simulink model "Algorithm"  (R2024a)
settings: Solver=FixedStepDiscrete  StartTime=0.0  StopTime=ALG_Stop_Time  FixedStep=ALG_Step_Size  RelTol=1e-3  EnableMultiTasking=on
undefined symbols (not defined in the file): BSD_WARN_DISTANCE_M, BSDState_T, RadarStatus_T, SignalStatus_T, TurnSignal_T, VSPD_SUPPRESSION_THRESHOLD
libraries: simulink x14
settings Model: DataDictionary=bsd.sldd  Creator=pc  LastModifiedBy=pc
settings OptimizationCC: DefaultParameterBehavior=Inlined  UseDivisionForNetSlopeComputation=on  EnhancedBackFolding=on  PassReuseOutputArgsAs=Individual arguments  ZeroExternalMemoryAtStartup=off  ZeroInternalMemoryAtStartup=off  OptimizeBlockOrder=speed  DifferentSizesBufferReuse=on  OptimizationCustomize=off  EfficientTunableParamExpr=on
settings DebuggingCC: ParameterTunabilityLossMsg=error
settings SFSimCC: MATLABDynamicMemAlloc=off
settings RTWCC: Description=AUTOSAR  SystemTargetFile=autosar.tlc  GenCodeOnly=on  TemplateMakefile=ert_default_tmf  DataTypeReplacement=CDataTypesFixedWidth
settings CodeAppCC: ForceParamTrailComments=on  IgnoreCustomStorageClasses=off  OperatorAnnotations=on  SimulinkDataObjDesc=on  SFDataObjDesc=on  InsertBlockDesc=on
settings STFCustomTargetCC: MultiwordLength=256  ParMdlRefBuildCompliant=on  CompOptLevelCompliant=on  IncludeMdlTerminateFcn=off  CombineOutputUpdateFcns=on  SuppressErrorStatus=on  ERTCustomFileBanners=on  SupportNonFinite=off  SupportComplex=off  SupportContinuousTime=off  SupportNonInlinedSFcns=off  RemoveResetFunc=on  MATLABClassNameForMDSCustomization=Simulink.SoftwareTarget.ERTCustomization  AutosarCompliant=on  GRTInterface=off  LookupTableObjectStructAxisOrder=2,1,3,4,...  LUTObjectStructOrderEvenSpacing=Size,Table,Breakpoints  SystemTargetFile=autosar.tlc
settings ERTTargetCC: TargetLangStandard=C99 (ISO)  ConcurrentExecutionCompliant=off  IncludeMdlTerminateFcn=off  SuppressErrorStatus=on  SupportNonFinite=off  SupportComplex=off  ModelStepFunctionPrototypeControlCompliant=off  CPPClassGenCompliant=off  AutosarCompliant=on  LookupTableObjectStructAxisOrder=2,1,3,4,...  LUTObjectStructOrderEvenSpacing=Size,Table,Breakpoints  InlinedParameterPlacement=NonHierarchical  ERTCustomFileTemplate=example_file_process.tlc  BooleanTrueId=TRUE  BooleanFalseId=FALSE

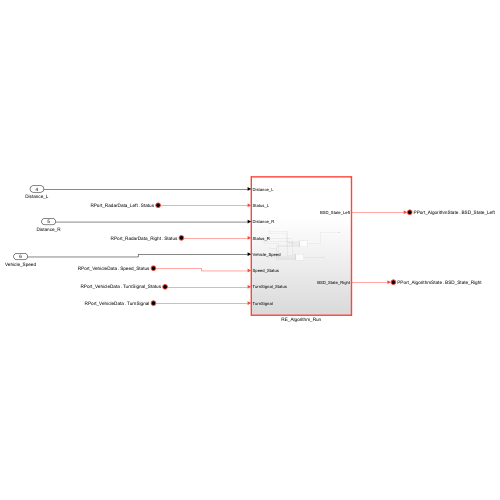
[thumbnail: Simulink's stored preview of the top-level diagram]
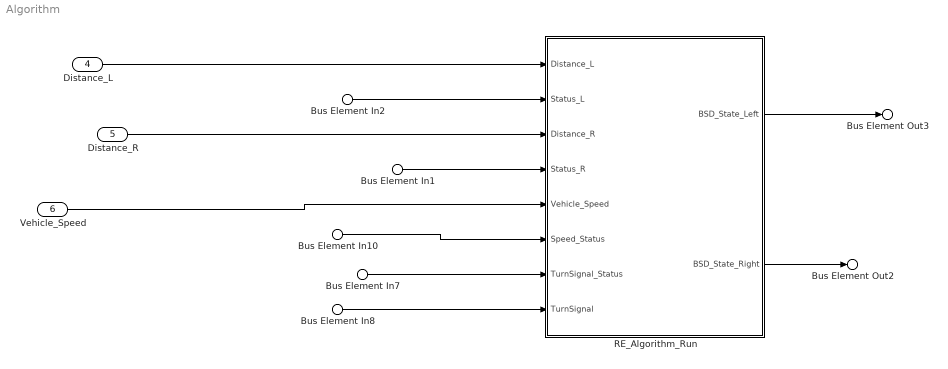
== system Algorithm ==
  Bus Element In7 : Inport  PortName=RPort_VehicleData  Element=TurnSignal_Status
  Bus Element In8 : Inport  PortName=RPort_VehicleData  Element=TurnSignal
  Bus Element In10 : Inport  PortName=RPort_VehicleData  Element=Speed_Status
  Bus Element In1 : Inport  Port=2  PortName=RPort_RadarData_Right  Element=Status
  Bus Element In2 : Inport  Port=3  PortName=RPort_RadarData_Left  Element=Status
  Distance_L : Inport  Port=4  OutDataTypeStr=Distance_m_T
  Distance_R : Inport  Port=5  OutDataTypeStr=Distance_m_T
  Vehicle_Speed : Inport  Port=6  OutDataTypeStr=Vehicle_Speed_T
  RE_Algorithm_Run : Subsystem  TreatAsAtomicUnit=on
  Bus Element Out2 : Outport  PortName=PPort_AlgorithmState  Element=BSD_State_Right
  Bus Element Out3 : Outport  PortName=PPort_AlgorithmState  Element=BSD_State_Left
  wires:
  Vehicle_Speed/1 -> RE_Algorithm_Run/5(Vehicle_Speed)
  Bus Element In10/1 -> RE_Algorithm_Run/6(Speed_Status)
  Bus Element In1/1 -> RE_Algorithm_Run/4(Status_R)
  Distance_L/1 -> RE_Algorithm_Run/1(Distance_L)
  Bus Element In2/1 -> RE_Algorithm_Run/2(Status_L)
  Distance_R/1 -> RE_Algorithm_Run/3(Distance_R)
  RE_Algorithm_Run/2(BSD_State_Right) -> Bus Element Out2/1
  RE_Algorithm_Run/1(BSD_State_Left) -> Bus Element Out3/1
  Bus Element In8/1 -> RE_Algorithm_Run/8(TurnSignal)
  Bus Element In7/1 -> RE_Algorithm_Run/7(TurnSignal_Status)

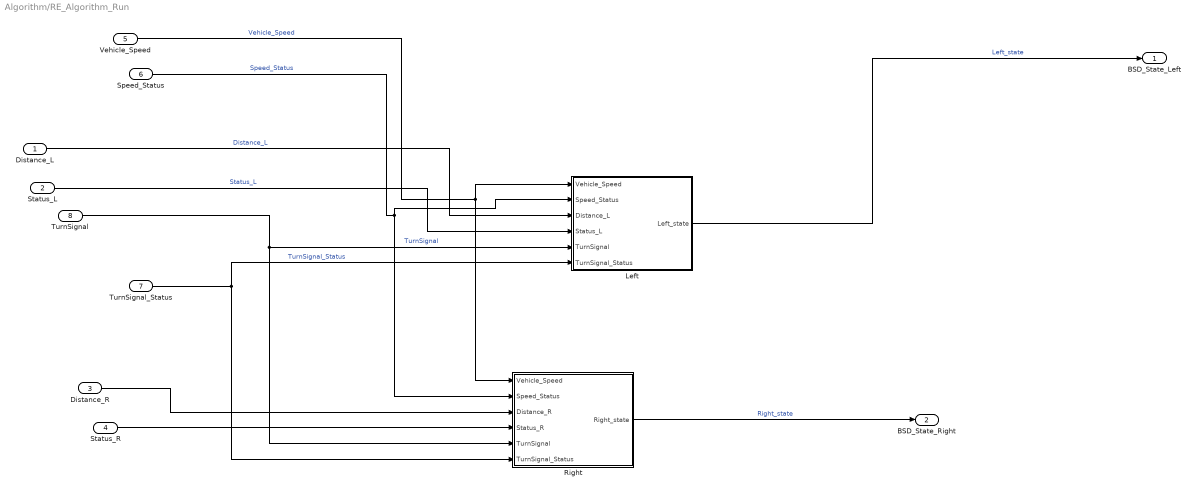
== system Algorithm/RE_Algorithm_Run ==
  Distance_L : Inport  OutDataTypeStr=Distance_m_T
  Status_L : Inport  Port=2  OutDataTypeStr=Enum: RadarStatus_T
  Distance_R : Inport  Port=3  OutDataTypeStr=Distance_m_T
  Status_R : Inport  Port=4  OutDataTypeStr=Enum: RadarStatus_T
  Vehicle_Speed : Inport  Port=5  OutDataTypeStr=Vehicle_Speed_T
  Speed_Status : Inport  Port=6  OutDataTypeStr=Enum: SignalStatus_T
  TurnSignal_Status : Inport  Port=7  OutDataTypeStr=Enum: SignalStatus_T
  TurnSignal : Inport  Port=8  OutDataTypeStr=Enum: TurnSignal_T
  Left : Subsystem
  Right : Subsystem
  BSD_State_Left : Outport  OutDataTypeStr=Enum: BSDState_T
  BSD_State_Right : Outport  Port=2  OutDataTypeStr=Enum: BSDState_T
  wires:
  Vehicle_Speed/1 -> Right/1(Vehicle_Speed), Left/1(Vehicle_Speed)  "Vehicle_Speed"
  Speed_Status/1 -> Right/2(Speed_Status), Left/2(Speed_Status)  "Speed_Status"
  Distance_L/1 -> Left/3(Distance_L)  "Distance_L"
  Status_L/1 -> Left/4(Status_L)  "Status_L"
  TurnSignal/1 -> Right/5(TurnSignal), Left/5(TurnSignal)  "TurnSignal"
  TurnSignal_Status/1 -> Left/6(TurnSignal_Status), Right/6(TurnSignal_Status)  "TurnSignal_Status"
  Left/1(Left_state) -> BSD_State_Left/1  "Left_state"
  Right/1(Right_state) -> BSD_State_Right/1  "Right_state"
  Distance_R/1 -> Right/3(Distance_R)
  Status_R/1 -> Right/4(Status_R)

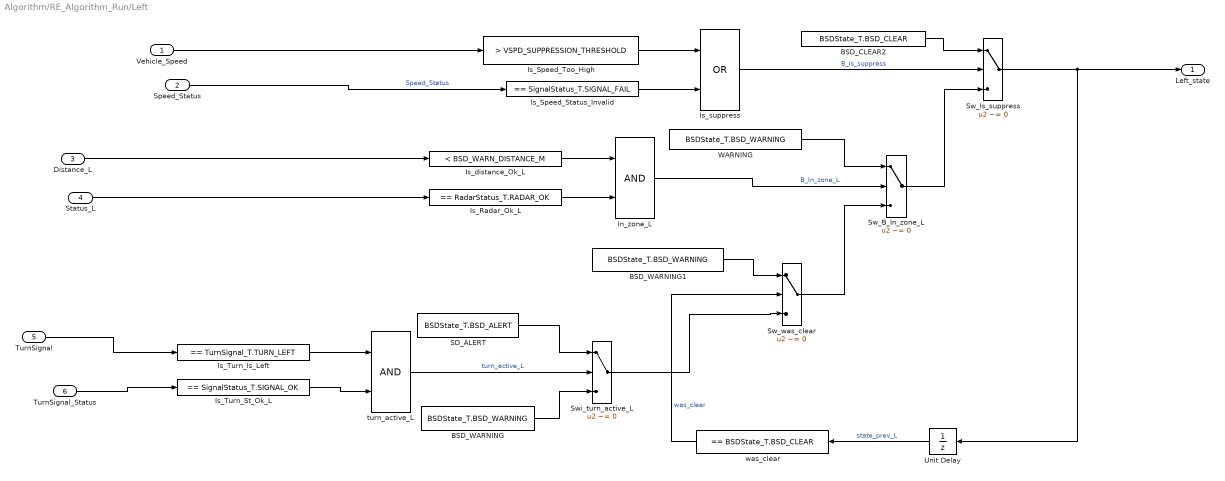
== system Algorithm/RE_Algorithm_Run/Left ==
  Vehicle_Speed : Inport  OutDataTypeStr=Vehicle_Speed_T
  Speed_Status : Inport  Port=2
  Distance_L : Inport  Port=3  OutDataTypeStr=Distance_m_T
  Status_L : Inport  Port=4
  TurnSignal : Inport  Port=5
  TurnSignal_Status : Inport  Port=6
  BSD_CLEAR2 : Constant  Value=BSDState_T.BSD_CLEAR  OutDataTypeStr=Enum: BSDState_T
  BSD_WARNING : Constant  Value=BSDState_T.BSD_WARNING  OutDataTypeStr=Enum: BSDState_T
  BSD_WARNING1 : Constant  Value=BSDState_T.BSD_WARNING  OutDataTypeStr=Enum: BSDState_T
  In_zone_L : Logic  AllPortsSameDT=off  OutDataTypeStr=boolean
  Is_Radar_Ok_L : simulink/Logic and Bit Operations/Compare To Constant  relop===  const=RadarStatus_T.RADAR_OK  OutDataTypeStr=boolean
  Is_Speed_Status_Invalid : simulink/Logic and Bit Operations/Compare To Constant  relop===  const=SignalStatus_T.SIGNAL_FAIL  OutDataTypeStr=boolean
  Is_Speed_Too_High : simulink/Logic and Bit Operations/Compare To Constant  relop=>  const=VSPD_SUPPRESSION_THRESHOLD  OutDataTypeStr=boolean
  Is_Turn_Is_Left : simulink/Logic and Bit Operations/Compare To Constant  relop===  const=TurnSignal_T.TURN_LEFT  OutDataTypeStr=boolean
  Is_Turn_St_Ok_L : simulink/Logic and Bit Operations/Compare To Constant  relop===  const=SignalStatus_T.SIGNAL_OK  OutDataTypeStr=boolean
  Is_distance_Ok_L : simulink/Logic and Bit Operations/Compare To Constant  relop=<  const=BSD_WARN_DISTANCE_M  OutDataTypeStr=boolean
  Is_suppress : Logic  Operator=OR  AllPortsSameDT=off  OutDataTypeStr=boolean
  SD_ALERT : Constant  Value=BSDState_T.BSD_ALERT  OutDataTypeStr=Enum: BSDState_T
  Sw_B_In_zone_L : Switch  Criteria=u2 ~= 0  SaturateOnIntegerOverflow=off  InputSameDT=off
  Sw_Is_suppress : Switch  Criteria=u2 ~= 0  SaturateOnIntegerOverflow=off  InputSameDT=off
  Sw_was_clear : Switch  Criteria=u2 ~= 0  SaturateOnIntegerOverflow=off  InputSameDT=off
  Swi_turn_active_L : Switch  Criteria=u2 ~= 0  SaturateOnIntegerOverflow=off  InputSameDT=off
  Unit Delay : UnitDelay  InitialCondition=BSDState_T.BSD_CLEAR  SampleTime=0.020  HasFrameUpgradeWarning=on
  WARNING : Constant  Value=BSDState_T.BSD_WARNING  OutDataTypeStr=Enum: BSDState_T
  turn_active_L : Logic  AllPortsSameDT=off  OutDataTypeStr=boolean
  was_clear : simulink/Logic and Bit Operations/Compare To Constant  relop===  const=BSDState_T.BSD_CLEAR  OutDataTypeStr=boolean
  Left_state : Outport
  wires:
  turn_active_L/1 -> Swi_turn_active_L/2  "turn_active_L"
  TurnSignal_Status/1 -> Is_Turn_St_Ok_L/1
  Is_Speed_Too_High/1 -> Is_suppress/1
  was_clear/1 -> Sw_was_clear/2  "was_clear"
  Is_Turn_St_Ok_L/1 -> turn_active_L/2
  BSD_WARNING1/1 -> Sw_was_clear/1
  Sw_Is_suppress/1 -> Left_state/1, Unit Delay/1
  Sw_was_clear/1 -> Sw_B_In_zone_L/3
  Is_Speed_Status_Invalid/1 -> Is_suppress/2
  Is_Turn_Is_Left/1 -> turn_active_L/1
  Is_distance_Ok_L/1 -> In_zone_L/1
  Speed_Status/1 -> Is_Speed_Status_Invalid/1  "Speed_Status"
  Is_Radar_Ok_L/1 -> In_zone_L/2
  Sw_B_In_zone_L/1 -> Sw_Is_suppress/3
  Status_L/1 -> Is_Radar_Ok_L/1
  In_zone_L/1 -> Sw_B_In_zone_L/2  "B_In_zone_L"
  Swi_turn_active_L/1 -> Sw_was_clear/3
  BSD_CLEAR2/1 -> Sw_Is_suppress/1
  Is_suppress/1 -> Sw_Is_suppress/2  "B_Is_suppress"
  Vehicle_Speed/1 -> Is_Speed_Too_High/1
  Unit Delay/1 -> was_clear/1  "state_prev_L"
  WARNING/1 -> Sw_B_In_zone_L/1
  BSD_WARNING/1 -> Swi_turn_active_L/3
  SD_ALERT/1 -> Swi_turn_active_L/1
  TurnSignal/1 -> Is_Turn_Is_Left/1
  Distance_L/1 -> Is_distance_Ok_L/1

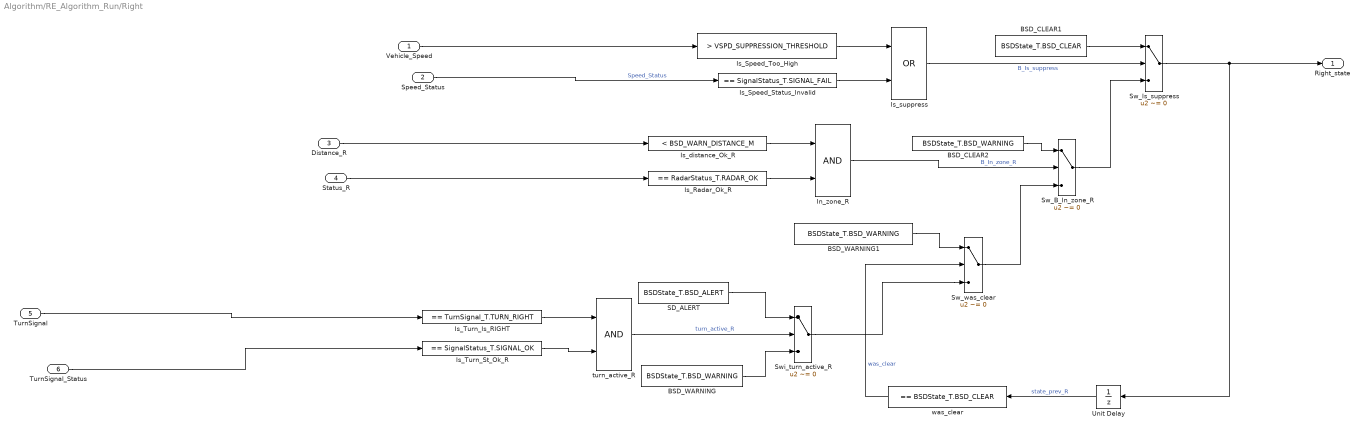
== system Algorithm/RE_Algorithm_Run/Right ==
  Vehicle_Speed : Inport
  Speed_Status : Inport  Port=2
  Distance_R : Inport  Port=3
  Status_R : Inport  Port=4
  TurnSignal : Inport  Port=5
  TurnSignal_Status : Inport  Port=6
  BSD_CLEAR1 : Constant  Value=BSDState_T.BSD_CLEAR  OutDataTypeStr=Enum: BSDState_T
  BSD_CLEAR2 : Constant  Value=BSDState_T.BSD_WARNING  OutDataTypeStr=Enum: BSDState_T
  BSD_WARNING : Constant  Value=BSDState_T.BSD_WARNING  OutDataTypeStr=Enum: BSDState_T
  BSD_WARNING1 : Constant  Value=BSDState_T.BSD_WARNING  OutDataTypeStr=Enum: BSDState_T
  In_zone_R : Logic  AllPortsSameDT=off  OutDataTypeStr=boolean
  Is_Radar_Ok_R : simulink/Logic and Bit Operations/Compare To Constant  relop===  const=RadarStatus_T.RADAR_OK  OutDataTypeStr=boolean
  Is_Speed_Status_Invalid : simulink/Logic and Bit Operations/Compare To Constant  relop===  const=SignalStatus_T.SIGNAL_FAIL  OutDataTypeStr=boolean
  Is_Speed_Too_High : simulink/Logic and Bit Operations/Compare To Constant  relop=>  const=VSPD_SUPPRESSION_THRESHOLD  OutDataTypeStr=boolean
  Is_Turn_Is_RIGHT : simulink/Logic and Bit Operations/Compare To Constant  relop===  const=TurnSignal_T.TURN_RIGHT  OutDataTypeStr=boolean
  Is_Turn_St_Ok_R : simulink/Logic and Bit Operations/Compare To Constant  relop===  const=SignalStatus_T.SIGNAL_OK  OutDataTypeStr=boolean
  Is_distance_Ok_R : simulink/Logic and Bit Operations/Compare To Constant  relop=<  const=BSD_WARN_DISTANCE_M  OutDataTypeStr=boolean
  Is_suppress : Logic  Operator=OR  AllPortsSameDT=off  OutDataTypeStr=boolean
  SD_ALERT : Constant  Value=BSDState_T.BSD_ALERT  OutDataTypeStr=Enum: BSDState_T
  Sw_B_In_zone_R : Switch  Criteria=u2 ~= 0  SaturateOnIntegerOverflow=off  InputSameDT=off
  Sw_Is_suppress : Switch  Criteria=u2 ~= 0  SaturateOnIntegerOverflow=off  InputSameDT=off
  Sw_was_clear : Switch  Criteria=u2 ~= 0  SaturateOnIntegerOverflow=off  InputSameDT=off
  Swi_turn_active_R : Switch  Criteria=u2 ~= 0  SaturateOnIntegerOverflow=off  InputSameDT=off
  Unit Delay : UnitDelay  InitialCondition=BSDState_T.BSD_CLEAR  SampleTime=0.020  HasFrameUpgradeWarning=on
  turn_active_R : Logic  AllPortsSameDT=off  OutDataTypeStr=boolean
  was_clear : simulink/Logic and Bit Operations/Compare To Constant  relop===  const=BSDState_T.BSD_CLEAR  OutDataTypeStr=boolean
  Right_state : Outport
  wires:
  Distance_R/1 -> Is_distance_Ok_R/1
  TurnSignal/1 -> Is_Turn_Is_RIGHT/1
  SD_ALERT/1 -> Swi_turn_active_R/1
  BSD_WARNING/1 -> Swi_turn_active_R/3
  Unit Delay/1 -> was_clear/1  "state_prev_R"
  Vehicle_Speed/1 -> Is_Speed_Too_High/1
  Is_suppress/1 -> Sw_Is_suppress/2  "B_Is_suppress"
  Swi_turn_active_R/1 -> Sw_was_clear/3
  In_zone_R/1 -> Sw_B_In_zone_R/2  "B_In_zone_R"
  Sw_B_In_zone_R/1 -> Sw_Is_suppress/3
  Is_Radar_Ok_R/1 -> In_zone_R/2
  Speed_Status/1 -> Is_Speed_Status_Invalid/1  "Speed_Status"
  Is_distance_Ok_R/1 -> In_zone_R/1
  Is_Turn_Is_RIGHT/1 -> turn_active_R/1
  Is_Speed_Status_Invalid/1 -> Is_suppress/2
  Sw_was_clear/1 -> Sw_B_In_zone_R/3
  Sw_Is_suppress/1 -> Unit Delay/1, Right_state/1
  BSD_WARNING1/1 -> Sw_was_clear/1
  Is_Turn_St_Ok_R/1 -> turn_active_R/2
  was_clear/1 -> Sw_was_clear/2  "was_clear"
  Is_Speed_Too_High/1 -> Is_suppress/1
  TurnSignal_Status/1 -> Is_Turn_St_Ok_R/1
  turn_active_R/1 -> Swi_turn_active_R/2  "turn_active_R"
  BSD_CLEAR1/1 -> Sw_Is_suppress/1
  BSD_CLEAR2/1 -> Sw_B_In_zone_R/1
  Status_R/1 -> Is_Radar_Ok_R/1
